simulink model "My_gfm_battery_sil_12_ConvIGBT_zDomain"  (R2025b)
settings: Solver=ode23t  StartTime=0.0  StopTime=10  MaxStep=1e-4  RelTol=1e-3
PreLoadFcn:
  | close all;
  | clear all;
  | clc;
  | 
  | 
  | modelDir = fileparts(get_param(bdroot,'FileName'));
  | 
  | load_system(fullfile(modelDir,'controls_element_lib.slx'));
  | load_system(fullfile(modelDir,'test_sequence_lib.slx'));
  | 
  | Simulink.importExternalCTypes('.\circuitControls\circuitControls_A_autogen.h')
InitFcn:
  | % frequency nominals
  | F_NOM = 60;
  | W_NOM = 2 * pi * F_NOM;
  | 
  | % base values relative to inverter
  | % --------------------------------
  | VLL_INV_NOM = 480;
  | P_INV_NOM = 1e6;
  | Q_INV_NOM = 0.5e6;
  | S_INV_NOM = sqrt(P_INV_NOM^2 + Q_INV_NOM^2);
  | 
  | I_INV_BASE = S_INV_NOM/(sqrt(3)*VLL_INV_NOM);
  | Z_INV_BASE = VLL_INV_NOM^2/S_INV_NOM;
  | L_INV_BASE = Z_INV_BASE / W_NOM;
  | C_INV_BASE = 1 / (Z_INV_BASE * W_NOM);
  | 
  | % nominal ratings for power system model
  | % --------------------------------------
  | INVERTER_COUNT = 100;
  | 
  | VLV_NOM = VLL_INV_NOM;
  | VMV_NOM = 35e3;
  | VHV_NOM = 230e3;
  | S_PLANT = INVERTER_COUNT * S_INV_NOM;
  | 
  | N_GSU = VHV_NOM/VMV_NOM;
  | N_MVT = VMV_NOM/VLV_NOM;
  | 
  | I_LV_BASE = S_PLANT/(sqrt(3)*VLV_NOM);
  | I_MV_BASE = S_PLANT/(sqrt(3)*VMV_NOM);
  | I_HV_BASE = S_PLANT/(sqrt(3)*VHV_NOM);
  | 
  | Z_LV_BASE = VLV_NOM^2/S_PLANT;
  | Z_MV_BASE = VMV_NOM^2/S_PLANT;
  | Z_HV_BASE = VHV_NOM^2/S_PLANT;
  | 
  | L_LV_BASE = Z_LV_BASE / W_NOM;
  | L_MV_BASE = Z_MV_BASE / W_NOM;
  | L_HV_BASE = Z_HV_BASE / W_NOM;
  | C_LV_BASE = 1 / (Z_LV_BASE * W_NOM);
  | C_MV_BASE = 1 / (Z_MV_BASE * W_NOM);
  | C_HV_BASE = 1 / (Z_HV_BASE * W_NOM);
undefined symbols (not defined in the file): D1, D11, Delta, gcbh, j, SampleTime, sps_rtmsupport, Ts
libraries: simulink x56, spsVoltageMeasurementLib x21, spsThreePhaseSeriesRLCBranchLib x20, spsControlledCurrentSourceLib x20, spsControlledVoltageSourceLib x15, spsThreePhaseVIMeasurementLib x12, spsSeriesRLCBranchLib x11, spsGroundLib x11, test_sequence_lib x10, controls_element_lib x8, spsCurrentMeasurementLib x8, spsThreePhaseTransformerTwoWindingsLib x6
(part 8 of 9)

== system My_gfm_battery_sil_12_ConvIGBT_zDomain/ac Network with MVT (native math)5/Network Interface1/CSI2 ==
  I : Inport
  Demux : Demux  Outputs=3
  Series RLC Branch : spsSeriesRLCBranchLib/Series RLC Branch  LConnTagsString=__new0  RConnTagsString=__new0  BranchType=R  Resistance=1e3  Inductance=1e-3  SetiL0=off  InitialCurrent=0  Capacitance=1e-6  Setx0=off  InitialVoltage=0  Measurements=None
  Series RLC Branch1 : spsSeriesRLCBranchLib/Series RLC Branch  LConnTagsString=__new0  RConnTagsString=__new0  BranchType=R  Resistance=1e3  Inductance=1e-3  SetiL0=off  InitialCurrent=0  Capacitance=1e-6  Setx0=off  InitialVoltage=0  Measurements=None
  Series RLC Branch2 : spsSeriesRLCBranchLib/Series RLC Branch  LConnTagsString=__new0  RConnTagsString=__new0  BranchType=R  Resistance=1e3  Inductance=1e-3  SetiL0=off  InitialCurrent=0  Capacitance=1e-6  Setx0=off  InitialVoltage=0  Measurements=None
  iA : spsControlledCurrentSourceLib/Controlled Current Source  Initialize=off  Source_Type=AC  Amplitude=0  Phase=0  Frequency=0  Measurements=None
  iB : spsControlledCurrentSourceLib/Controlled Current Source  Initialize=off  Source_Type=AC  Amplitude=0  Phase=0  Frequency=0  Measurements=None
  iB1 : spsControlledCurrentSourceLib/Controlled Current Source  Initialize=off  Source_Type=AC  Amplitude=0  Phase=0  Frequency=0  Measurements=None
  A : PMIOPort  Side=Right
  B : PMIOPort  Port=2  Side=Right
  C : PMIOPort  Port=3  Side=Right
  wires:
  Demux/1 -> iA/1
  Demux/2 -> iB/1
  I/1 -> Demux/1
  Demux/3 -> iB1/1
  connections:
  iA/RConn1 -- A/RConn1 -- Series RLC Branch/LConn1
  iB/RConn1 -- B/RConn1 -- Series RLC Branch1/LConn1
  Series RLC Branch1/RConn1 -- Series RLC Branch/RConn1 -- iA/LConn1 -- iB/LConn1 -- iB1/LConn1 -- Series RLC Branch2/RConn1
  C/RConn1 -- iB1/RConn1 -- Series RLC Branch2/LConn1

== system My_gfm_battery_sil_12_ConvIGBT_zDomain/ac Network with MVT (native math)5/Network Interface1/Cur Meas ==
  Current Measurement : spsCurrentMeasurementLib/Current Measurement  PhasorSimulation=off  OutputType=Complex  PSBequivalent=0
  Current Measurement1 : spsCurrentMeasurementLib/Current Measurement  PhasorSimulation=off  OutputType=Complex  PSBequivalent=0
  Current Measurement2 : spsCurrentMeasurementLib/Current Measurement  PhasorSimulation=off  OutputType=Complex  PSBequivalent=0
  Mux : Mux  Inputs=3
  A : PMIOPort  Side=Left
  B : PMIOPort  Port=2  Side=Left
  C : PMIOPort  Port=3  Side=Left
  a : PMIOPort  Port=4  Side=Right
  b : PMIOPort  Port=5  Side=Right
  c : PMIOPort  Port=6  Side=Right
  I : Outport  VectorParamsAs1DForOutWhenUnconnected=off
  wires:
  Current Measurement/1 -> Mux/1
  Current Measurement1/1 -> Mux/2
  Mux/1 -> I/1
  Current Measurement2/1 -> Mux/3
  connections:
  Current Measurement1/LConn1 -- B/RConn1
  Current Measurement/LConn1 -- A/RConn1
  Current Measurement2/LConn1 -- C/RConn1
  a/RConn1 -- Current Measurement/RConn1
  b/RConn1 -- Current Measurement1/RConn1
  c/RConn1 -- Current Measurement2/RConn1

== system My_gfm_battery_sil_12_ConvIGBT_zDomain/ac Network with MVT (native math)5/Network Interface1/Subsystem ==
  In1 : Inport
  Demux : Demux  Outputs=3
  Mux : Mux  Inputs=3
  Transfer Fcn : TransferFcn  Denominator=[1e-6 1]
  Transfer Fcn1 : TransferFcn  Denominator=[1e-6 1]
  Transfer Fcn2 : TransferFcn  Denominator=[1e-6 1]
  Out1 : Outport  VectorParamsAs1DForOutWhenUnconnected=off
  wires:
  Demux/2 -> Transfer Fcn2/1
  Demux/1 -> Transfer Fcn/1
  Transfer Fcn1/1 -> Mux/3
  Mux/1 -> Out1/1
  Transfer Fcn2/1 -> Mux/2
  Demux/3 -> Transfer Fcn1/1
  Transfer Fcn/1 -> Mux/1
  In1/1 -> Demux/1

== system My_gfm_battery_sil_12_ConvIGBT_zDomain/ac Network with MVT (native math)5/Network Interface1/Subsystem1 ==
  In1 : Inport
  Demux : Demux  Outputs=3
  Mux : Mux  Inputs=3
  Transfer Fcn : TransferFcn  Denominator=[1e-6 1]
  Transfer Fcn1 : TransferFcn  Denominator=[1e-6 1]
  Transfer Fcn2 : TransferFcn  Denominator=[1e-6 1]
  Out1 : Outport  VectorParamsAs1DForOutWhenUnconnected=off
  wires:
  Demux/2 -> Transfer Fcn2/1
  Demux/1 -> Transfer Fcn/1
  Transfer Fcn1/1 -> Mux/3
  Mux/1 -> Out1/1
  Transfer Fcn2/1 -> Mux/2
  Demux/3 -> Transfer Fcn1/1
  Transfer Fcn/1 -> Mux/1
  In1/1 -> Demux/1

== system My_gfm_battery_sil_12_ConvIGBT_zDomain/ac Network with MVT (native math)5/Network Interface1/VSI1 ==
  V : Inport
  Controlled Voltage Source : spsControlledVoltageSourceLib/Controlled Voltage Source  Initialize=off  Source_Type=AC  Amplitude=0  Phase=0  Frequency=0  Measurements=None
  Controlled Voltage Source1 : spsControlledVoltageSourceLib/Controlled Voltage Source  Initialize=off  Source_Type=AC  Amplitude=0  Phase=0  Frequency=0  Measurements=None
  Demux : Demux  Outputs=3
  Terminator : Terminator
  A : PMIOPort  Side=Right
  B : PMIOPort  Port=2  Side=Right
  C : PMIOPort  Port=3  Side=Right
  wires:
  Demux/1 -> Controlled Voltage Source/1
  Demux/2 -> Controlled Voltage Source1/1
  V/1 -> Demux/1
  Demux/3 -> Terminator/1
  connections:
  Controlled Voltage Source/RConn1 -- A/RConn1
  Controlled Voltage Source1/RConn1 -- B/RConn1
  Controlled Voltage Source1/LConn1 -- Controlled Voltage Source/LConn1 -- C/RConn1

== system My_gfm_battery_sil_12_ConvIGBT_zDomain/ac Network with MVT (native math)5/Network Interface1/Volt Meas1 ==
  Ground : Ground
  Mux : Mux  Inputs=3
  V_AB : spsVoltageMeasurementLib/Voltage Measurement  PhasorSimulation=off  OutputType=Complex  PSBequivalent=0
  V_BC : spsVoltageMeasurementLib/Voltage Measurement  PhasorSimulation=off  OutputType=Complex  PSBequivalent=0
  A : PMIOPort  Side=Left
  B : PMIOPort  Port=2  Side=Left
  C : PMIOPort  Port=3  Side=Left
  V : Outport  VectorParamsAs1DForOutWhenUnconnected=off
  wires:
  V_AB/1 -> Mux/1
  V_BC/1 -> Mux/2
  Mux/1 -> V/1  "[Vab,Vbc]"
  Ground/1 -> Mux/3
  connections:
  V_BC/LConn1 -- B/RConn1
  A/RConn1 -- V_AB/LConn1
  C/RConn1 -- V_AB/LConn2 -- V_BC/LConn2

== system My_gfm_battery_sil_12_ConvIGBT_zDomain/ac Network with MVT (native math)5/Two-Level Converter/Model1 ==
  note: (Uref)
  g : Inport  SampleTime=Ts
  Block : Inport  Port=2
  Add : Sum  Inputs=+-
  Constant : Constant
  Constant1 : Constant  Value=0
  Constant2 : Constant
  Current Measurement : spsCurrentMeasurementLib/Current Measurement  PhasorSimulation=off  OutputType=Complex  PSBequivalent=0
  Data Type Conversion2 : DataTypeConversion  OutDataTypeStr=double  SaturateOnIntegerOverflow=off  RndMeth=Floor
  Demux : Demux  Outputs=2
  Fcn2 : Fcn  Expr=(u(1)+1)*0.5
  MATLAB Function : MATLAB Function  TreatAsAtomicUnit=on
  Mux : Mux  Inputs=2
  Mux1 : Mux  Inputs=2
  Power : spsHalfBridgeModel/Power  SystemSampleTime=-1  VariantActivationTime=update diagram  EmptyChoice=off  PassThrough=off  PassThroughVariantControl=(default)  EmptyChoiceVariantControl=(default)  AllowFlexibleInterface=on  Latency=0  AutoFrameSizeCalculation=off
  Product2 : Product
  Product8 : Product
  Saturation : Saturate  UpperLimit=1.0  LowerLimit=-1.0
  Scope : Scope  NumInputPorts=2
      settings: ActiveDisplayYMinimum=-0.125  ActiveDisplayYMaximum=1.125
  Scope1 : Scope  NumInputPorts=2
      settings: ActiveDisplayYMinimum=0.0581  ActiveDisplayYMaximum=0.93277  DataLoggingVariableName=ScopeData2
  Scope2 : Scope  NumInputPorts=6
      settings: ActiveDisplayYMinimum=-1057.03298  ActiveDisplayYMaximum=1237.20421  DataLoggingVariableName=ScopeData3
  Switch : Switch  Criteria=u2 > Threshold  SaturateOnIntegerOverflow=off  InputSameDT=off
  Transfer Fcn : TransferFcn  Denominator=[1e-6 1]
  Transfer Fcn1 : TransferFcn  Denominator=[1e-6 1]
  Transfer Fcn2 : TransferFcn  Denominator=[1e-6 1]
  Voltage Measurement : spsVoltageMeasurementLib/Voltage Measurement  PhasorSimulation=off  OutputType=Complex  PSBequivalent=0
  + : PMIOPort  Tag=PMCPort  Side=Right
  - : PMIOPort  Tag=PMCPort  Port=2  Side=Right
  Out : PMIOPort  Tag=PMCPort  Port=3  Side=Left
  wires:
  Saturation/1 -> Fcn2/1
  g/1 -> Saturation/1
  Block/1 -> Switch/2, Scope/1
  Data Type Conversion2/1 -> Scope/2, Product2/1, Product8/1
  Product2/1 -> Mux1/1
  Product8/1 -> Mux1/2
  Add/1 -> Scope1/2, Product8/2
  Constant/1 -> Add/1
  Fcn2/1 -> Add/2, Scope1/1, Product2/2
  Switch/1 -> Data Type Conversion2/1
  Power/2 -> Scope2/4, Demux/1
  Demux/2 -> Transfer Fcn2/1
  Demux/1 -> Transfer Fcn/1
  Transfer Fcn/1 -> Mux/1
  Transfer Fcn2/1 -> Mux/2
  Mux/1 -> MATLAB Function/3(I)
  Transfer Fcn1/1 -> MATLAB Function/2(Vdc)
  Power/1 -> Scope2/2, Transfer Fcn1/1
  MATLAB Function/2(Idc) -> Power/2, Scope2/3
  MATLAB Function/1(V) -> Power/1, Scope2/1
  Mux1/1 -> MATLAB Function/1(g)
  Constant1/1 -> Switch/1
  Constant2/1 -> Switch/3
  Voltage Measurement/1 -> Scope2/5
  Current Measurement/1 -> Scope2/6
  connections:
  Power/LConn1 -- Current Measurement/LConn1 -- Voltage Measurement/LConn1
  Power/RConn2 -- Voltage Measurement/LConn2 -- -/RConn1
  Power/RConn1 -- +/RConn1
  Current Measurement/RConn1 -- Out/RConn1

== system My_gfm_battery_sil_12_ConvIGBT_zDomain/ac Network with MVT (native math)5/Two-Level Converter/Model2 ==
  note: (Uref)
  g : Inport  SampleTime=Ts
  Block : Inport  Port=2
  Add : Sum  Inputs=+-
  Constant : Constant
  Constant1 : Constant  Value=0
  Constant2 : Constant
  Data Type Conversion2 : DataTypeConversion  OutDataTypeStr=double  SaturateOnIntegerOverflow=off  RndMeth=Floor
  Demux : Demux  Outputs=2
  Fcn2 : Fcn  Expr=(u(1)+1)*0.5
  MATLAB Function : MATLAB Function  TreatAsAtomicUnit=on
  Mux : Mux  Inputs=2
  Mux1 : Mux  Inputs=2
  Power : spsHalfBridgeModel/Power  SystemSampleTime=-1  VariantActivationTime=update diagram  EmptyChoice=off  PassThrough=off  PassThroughVariantControl=(default)  EmptyChoiceVariantControl=(default)  AllowFlexibleInterface=on  Latency=0  AutoFrameSizeCalculation=off
  Product2 : Product
  Product8 : Product
  Saturation : Saturate  UpperLimit=1.0  LowerLimit=-1.0
  Scope : Scope  NumInputPorts=2
      settings: ActiveDisplayYMinimum=-0.125  ActiveDisplayYMaximum=1.125
  Scope1 : Scope  NumInputPorts=2
      settings: ActiveDisplayYMinimum=-0.0256  ActiveDisplayYMaximum=0.96024  DataLoggingVariableName=ScopeData2
  Scope2 : Scope  NumInputPorts=5
      settings: ActiveDisplayYMinimum=-1250  ActiveDisplayYMaximum=1079.00943  DataLoggingVariableName=ScopeData3
  Switch : Switch  Criteria=u2 > Threshold  SaturateOnIntegerOverflow=off  InputSameDT=off
  Transfer Fcn : TransferFcn  Denominator=[1e-6 1]
  Transfer Fcn1 : TransferFcn  Denominator=[1e-6 1]
  Transfer Fcn2 : TransferFcn  Denominator=[1e-6 1]
  Voltage Measurement : spsVoltageMeasurementLib/Voltage Measurement  PhasorSimulation=off  OutputType=Complex  PSBequivalent=0
  + : PMIOPort  Tag=PMCPort  Side=Right
  - : PMIOPort  Tag=PMCPort  Port=2  Side=Right
  Out : PMIOPort  Tag=PMCPort  Port=3  Side=Left
  wires:
  Saturation/1 -> Fcn2/1
  g/1 -> Saturation/1
  Block/1 -> Switch/2, Scope/1
  Data Type Conversion2/1 -> Scope/2, Product2/1, Product8/1
  Product2/1 -> Mux1/1
  Product8/1 -> Mux1/2
  Add/1 -> Scope1/2, Product8/2
  Constant/1 -> Add/1
  Fcn2/1 -> Add/2, Scope1/1, Product2/2
  Switch/1 -> Data Type Conversion2/1
  Power/2 -> Scope2/4, Demux/1
  Demux/2 -> Transfer Fcn2/1
  Demux/1 -> Transfer Fcn/1
  Transfer Fcn/1 -> Mux/1
  Transfer Fcn2/1 -> Mux/2
  Mux/1 -> MATLAB Function/3(I)
  Transfer Fcn1/1 -> MATLAB Function/2(Vdc)
  Power/1 -> Scope2/2, Transfer Fcn1/1
  MATLAB Function/2(Idc) -> Power/2, Scope2/3
  MATLAB Function/1(V) -> Power/1, Scope2/1
  Mux1/1 -> MATLAB Function/1(g)
  Constant1/1 -> Switch/1
  Constant2/1 -> Switch/3
  Voltage Measurement/1 -> Scope2/5
  connections:
  Out/RConn1 -- Power/LConn1 -- Voltage Measurement/LConn1
  -/RConn1 -- Power/RConn2 -- Voltage Measurement/LConn2
  Power/RConn1 -- +/RConn1

== system My_gfm_battery_sil_12_ConvIGBT_zDomain/ac Network with MVT (native math)5/Two-Level Converter/Model3 ==
  note: (Uref)
  g : Inport  SampleTime=Ts
  Block : Inport  Port=2
  Add : Sum  Inputs=+-
  Constant : Constant
  Constant1 : Constant  Value=0
  Constant2 : Constant
  Data Type Conversion2 : DataTypeConversion  OutDataTypeStr=double  SaturateOnIntegerOverflow=off  RndMeth=Floor
  Demux : Demux  Outputs=2
  Fcn2 : Fcn  Expr=(u(1)+1)*0.5
  MATLAB Function : MATLAB Function  TreatAsAtomicUnit=on
  Mux : Mux  Inputs=2
  Mux1 : Mux  Inputs=2
  Power : spsHalfBridgeModel/Power  SystemSampleTime=-1  VariantActivationTime=update diagram  EmptyChoice=off  PassThrough=off  PassThroughVariantControl=(default)  EmptyChoiceVariantControl=(default)  AllowFlexibleInterface=on  Latency=0  AutoFrameSizeCalculation=off
  Product2 : Product
  Product8 : Product
  Saturation : Saturate  UpperLimit=1.0  LowerLimit=-1.0
  Scope : Scope  NumInputPorts=2
      settings: ActiveDisplayYMinimum=-0.125  ActiveDisplayYMaximum=1.125
  Scope1 : Scope  NumInputPorts=2
      settings: ActiveDisplayYMinimum=-0.0256  ActiveDisplayYMaximum=0.96024  DataLoggingVariableName=ScopeData2
  Scope2 : Scope  NumInputPorts=5
      settings: ActiveDisplayYMinimum=-1250  ActiveDisplayYMaximum=1079.00943  DataLoggingVariableName=ScopeData3
  Switch : Switch  Criteria=u2 > Threshold  SaturateOnIntegerOverflow=off  InputSameDT=off
  Transfer Fcn : TransferFcn  Denominator=[1e-6 1]
  Transfer Fcn1 : TransferFcn  Denominator=[1e-6 1]
  Transfer Fcn2 : TransferFcn  Denominator=[1e-6 1]
  Voltage Measurement : spsVoltageMeasurementLib/Voltage Measurement  PhasorSimulation=off  OutputType=Complex  PSBequivalent=0
  + : PMIOPort  Tag=PMCPort  Side=Right
  - : PMIOPort  Tag=PMCPort  Port=2  Side=Right
  Out : PMIOPort  Tag=PMCPort  Port=3  Side=Left
  wires:
  Saturation/1 -> Fcn2/1
  g/1 -> Saturation/1
  Block/1 -> Switch/2, Scope/1
  Data Type Conversion2/1 -> Scope/2, Product2/1, Product8/1
  Product2/1 -> Mux1/1
  Product8/1 -> Mux1/2
  Add/1 -> Scope1/2, Product8/2
  Constant/1 -> Add/1
  Fcn2/1 -> Add/2, Scope1/1, Product2/2
  Switch/1 -> Data Type Conversion2/1
  Power/2 -> Scope2/4, Demux/1
  Demux/2 -> Transfer Fcn2/1
  Demux/1 -> Transfer Fcn/1
  Transfer Fcn/1 -> Mux/1
  Transfer Fcn2/1 -> Mux/2
  Mux/1 -> MATLAB Function/3(I)
  Transfer Fcn1/1 -> MATLAB Function/2(Vdc)
  Power/1 -> Scope2/2, Transfer Fcn1/1
  MATLAB Function/2(Idc) -> Power/2, Scope2/3
  MATLAB Function/1(V) -> Power/1, Scope2/1
  Mux1/1 -> MATLAB Function/1(g)
  Constant1/1 -> Switch/1
  Constant2/1 -> Switch/3
  Voltage Measurement/1 -> Scope2/5
  connections:
  Out/RConn1 -- Power/LConn1 -- Voltage Measurement/LConn1
  -/RConn1 -- Power/RConn2 -- Voltage Measurement/LConn2
  Power/RConn1 -- +/RConn1

== system My_gfm_battery_sil_12_ConvIGBT_zDomain/My Inverter Controller /My_acMonitor_A/Analyzer_V/complex_LPF ==
  note: This was needed because Simulink complains when using transfer functions directly on arrays or complex numbers.
  In1 : Inport
  Complex to Real-Imag : ComplexToRealImag
  LPF1 : Subsystem  SystemSampleTime=1/20000  mask(Low Pass Filter){Ts=Ts, OmegaUp=1/tau, OmegaDn=1/tau}
      mask prompts: Ts "Tsample"; OmegaUp "Up Path Bandwidth"; OmegaDn "Down Path Bandwidth"
  LPF4 : Subsystem  SystemSampleTime=1/20000  mask(Low Pass Filter){Ts=Ts, OmegaUp=1/tau, OmegaDn=1/tau}
      mask prompts: Ts "Tsample"; OmegaUp "Up Path Bandwidth"; OmegaDn "Down Path Bandwidth"
  Real-Imag to Complex : RealImagToComplex
  Out1 : Outport
  wires:
  Real-Imag to Complex/1 -> Out1/1
  In1/1 -> Complex to Real-Imag/1
  Complex to Real-Imag/1 -> LPF4/1(in)
  LPF4/1(out) -> Real-Imag to Complex/1
  Complex to Real-Imag/2 -> LPF1/1(in)
  LPF1/1(out) -> Real-Imag to Complex/2

== system My_gfm_battery_sil_12_ConvIGBT_zDomain/My Inverter Controller /My_acMonitor_A/Analyzer_V1/complex_LPF ==
  note: This was needed because Simulink complains when using transfer functions directly on arrays or complex numbers.
  In1 : Inport
  Complex to Real-Imag : ComplexToRealImag
  Gain2 : Gain  Gain=1/tau
  Gain3 : Gain  Gain=1/tau
  Integrator : Integrator
  Integrator1 : Integrator
  Real-Imag to Complex : RealImagToComplex
  Sum : Sum  Inputs=|+-
  Sum1 : Sum  Inputs=|+-
  Out1 : Outport
  wires:
  Real-Imag to Complex/1 -> Out1/1
  In1/1 -> Complex to Real-Imag/1
  Complex to Real-Imag/1 -> Sum/1
  Integrator/1 -> Real-Imag to Complex/1, Sum/2
  Sum1/1 -> Gain3/1
  Complex to Real-Imag/2 -> Sum1/1
  Gain2/1 -> Integrator/1
  Sum/1 -> Gain2/1
  Integrator1/1 -> Sum1/2, Real-Imag to Complex/2
  Gain3/1 -> Integrator1/1

== system My_gfm_battery_sil_12_ConvIGBT_zDomain/My Inverter Controller /My_acMonitor_A/PLL_3ph1/Integrator ==
  in : Inport
  rst : Inport  Port=2
  Constant : Constant  Value=0
  Constant1 : Constant  Value=HiLim
  Constant2 : Constant  Value=LoLim
  Constant3 : Constant  Value=Ts
  Delay : Delay  DelayLength=1  InitialCondition=0
  Logical Operator : Logic  Operator=NOT  AllPortsSameDT=off  OutDataTypeStr=boolean
  Product : Product
  Saturation Dynamic : simulink/Discontinuities/Saturation Dynamic  OutMin=[]  OutMax=[]  OutDataTypeStr=Inherit: Same as second input  OutDataType=fixdt(1, 16)  OutScaling=2^-10  DoSatur=off
  Sum : Sum  Inputs=|++
  Switch : Switch  Criteria=u2 ~= 0  SaturateOnIntegerOverflow=off  InputSameDT=off
  out : Outport
  FB : Outport  Port=2
  wires:
  Delay/1 -> Sum/2, FB/1
  Switch/1 -> Saturation Dynamic/2
  in/1 -> Product/2
  Product/1 -> Sum/1
  Constant3/1 -> Product/1
  Sum/1 -> Switch/1
  Constant/1 -> Switch/3
  rst/1 -> Logical Operator/1
  Logical Operator/1 -> Switch/2
  Saturation Dynamic/1 -> out/1, Delay/1
  Constant1/1 -> Saturation Dynamic/1
  Constant2/1 -> Saturation Dynamic/3

== system My_gfm_battery_sil_12_ConvIGBT_zDomain/My Inverter Controller /My_acMonitor_A/PLL_3ph1/LPF4 ==
  note: Forward integrator
  in : Inport
  Constant : Constant  Value=Ts
  Constant1 : Constant  Value=Ts
  Constant2 : Constant  Value=OmegaUp
  Constant3 : Constant  Value=OmegaUp
  Constant4 : Constant  Value=OmegaDn
  Delay : Delay  DelayLength=1  InitialCondition=0
  Product{,1..4} (5 alike) : Product
  Saturation : Saturate  UpperLimit=inf  LowerLimit=0
  Saturation1 : Saturate  UpperLimit=0  LowerLimit=-inf
  Sum : Sum  Inputs=|++
  Sum1 : Sum  Inputs=|++
  Sum4 : Sum  Inputs=|+-
  out : Outport
  wires:
  Delay/1 -> Sum4/2, Sum/2
  in/1 -> Sum4/1, Product4/2
  Sum4/1 -> Product2/1, Product1/2
  Sum/1 -> out/1, Delay/1
  Saturation/1 -> Sum1/1
  Saturation1/1 -> Sum1/2
  Sum1/1 -> Product/2
  Product/1 -> Sum/1
  Constant/1 -> Product/1
  Constant3/1 -> Product1/1
  Constant4/1 -> Product2/2
  Product1/1 -> Saturation/1
  Product2/1 -> Saturation1/1
  Product4/1 -> Product3/2
  Constant1/1 -> Product3/1
  Constant2/1 -> Product4/1

== system My_gfm_battery_sil_12_ConvIGBT_zDomain/My Inverter Controller /My_acMonitor_A/PLL_3ph1/SOGI1 ==
  in : Inport
  f : Inport  Port=2
  Gain : Gain
  Gain1 : Gain  Gain=alpha
  Gain2 : Gain  Gain=2*pi
  Ground : Ground
  Ground1 : Ground
  Integrator : Subsystem  SystemSampleTime=1/20000  mask(Limited Integrator){Ts=Ts, HiLim=inf, LoLim=-inf}
      mask prompts: Ts "Tsample"; HiLim "Integrator Upper Limiter"; LoLim "Integrator Lower Limiter"
  Integrator1 : Subsystem  SystemSampleTime=1/20000  mask(Limited Integrator){Ts=Ts, HiLim=inf, LoLim=-inf}
      mask prompts: Ts "Tsample"; HiLim "Integrator Upper Limiter"; LoLim "Integrator Lower Limiter"
  Product : Product
  Product2 : Product
  Sum : Sum  Inputs=|+-
  Sum1 : Sum  Inputs=|+-
  Sum2 : Sum  Inputs=|+-
  Terminator : Terminator
  Notched : Outport
  BandPassed : Outport  Port=2
  wires:
  f/1 -> Gain2/1
  in/1 -> Sum2/1, Sum1/1
  Integrator1/2(FB) -> Product2/1
  Gain/1 -> Sum1/2
  Sum1/1 -> Gain1/1
  Integrator/1(out) -> Integrator1/1(in), BandPassed/1
  Gain2/1 -> Product/2, Product2/2
  Sum/1 -> Product/1
  Product2/1 -> Sum/2
  Product/1 -> Integrator/1(in)
  Integrator/2(FB) -> Sum2/2, Gain/1
  Sum2/1 -> Notched/1
  Ground/1 -> Integrator/2(rst)
  Ground1/1 -> Integrator1/2(rst)
  Integrator1/1(out) -> Terminator/1
  Gain1/1 -> Sum/1

== system My_gfm_battery_sil_12_ConvIGBT_zDomain/My Inverter Controller /My_acMonitor_A/PLL_3ph1/oscillator_3ph ==
  f : Inport
  Cos : Trigonometry  Operator=cos
  Delay : Delay  DelayLength=1  InitialCondition=0
  Gain : Gain  Gain=2*pi
  Ground1 : Ground
  Integrator : Subsystem  SystemSampleTime=1/20000  mask(Wrapped Integrator){Ts=Ts}
      mask prompts: Ts "Tsample"
      mask help: output range : [0 to 1]
  Real-Imag to Complex : RealImagToComplex
  Scope : Scope
      settings: ActiveDisplayYMinimum=-0.026446027315415011  ActiveDisplayYMaximum=1.0606778639513765  DataLoggingVariableName=ScopeData13
  Sin : Trigonometry
  Sum1 : Sum  Inputs=|++
  Terminator : Terminator
  phase_shift : Constant  Value=[0 -1/3 -2/3]
  osc[3] : Outport
  osc[3]_FB : Outport  Port=2
  wires:
  Sum1/1 -> Gain/1
  phase_shift/1 -> Sum1/2
  Sin/1 -> Real-Imag to Complex/2
  Gain/1 -> Sin/1, Cos/1
  Cos/1 -> Real-Imag to Complex/1
  Real-Imag to Complex/1 -> Delay/1, osc[3]/1
  f/1 -> Integrator/1(in)
  Delay/1 -> osc[3]_FB/1
  Integrator/2(FB) -> Terminator/1
  Ground1/1 -> Integrator/2(rst)
  Integrator/1(out) -> Scope/1, Sum1/1

== system My_gfm_battery_sil_12_ConvIGBT_zDomain/My Inverter Controller /My_acMonitor_A/PLL_3ph2/oscillator_3ph ==
  f : Inport
  Cos : Trigonometry  Operator=cos
  Gain : Gain  Gain=2*pi
  Integrator : Integrator
  Real-Imag to Complex : RealImagToComplex
  Sin : Trigonometry
  Sum1 : Sum  Inputs=|++
  phase_shift : Constant  Value=[0 -1/3 -2/3]
  osc[3] : Outport
  wires:
  Sum1/1 -> Gain/1
  phase_shift/1 -> Sum1/2
  Sin/1 -> Real-Imag to Complex/2
  Integrator/1 -> Sum1/1
  Gain/1 -> Sin/1, Cos/1
  Cos/1 -> Real-Imag to Complex/1
  Real-Imag to Complex/1 -> osc[3]/1
  f/1 -> Integrator/1

== system My_gfm_battery_sil_12_ConvIGBT_zDomain/My Inverter Controller /My_acMonitor_A/RMS_Analyzer/LPF4 ==
  note: Forward integrator
  in : Inport
  Constant : Constant  Value=Ts
  Constant1 : Constant  Value=Ts
  Constant2 : Constant  Value=OmegaUp
  Constant3 : Constant  Value=OmegaUp
  Constant4 : Constant  Value=OmegaDn
  Delay : Delay  DelayLength=1  InitialCondition=0
  Product{,1..4} (5 alike) : Product
  Saturation : Saturate  UpperLimit=inf  LowerLimit=0
  Saturation1 : Saturate  UpperLimit=0  LowerLimit=-inf
  Sum : Sum  Inputs=|++
  Sum1 : Sum  Inputs=|++
  Sum4 : Sum  Inputs=|+-
  out : Outport
  wires:
  Delay/1 -> Sum4/2, Sum/2
  in/1 -> Sum4/1, Product4/2
  Sum4/1 -> Product2/1, Product1/2
  Sum/1 -> out/1, Delay/1
  Saturation/1 -> Sum1/1
  Saturation1/1 -> Sum1/2
  Sum1/1 -> Product/2
  Product/1 -> Sum/1
  Constant/1 -> Product/1
  Constant3/1 -> Product1/1
  Constant4/1 -> Product2/2
  Product1/1 -> Saturation/1
  Product2/1 -> Saturation1/1
  Product4/1 -> Product3/2
  Constant1/1 -> Product3/1
  Constant2/1 -> Product4/1

== system My_gfm_battery_sil_12_ConvIGBT_zDomain/My Inverter Controller /My_acMonitor_A/SOGI1/Integrator ==
  in : Inport
  rst : Inport  Port=2
  Constant : Constant  Value=0
  Constant1 : Constant  Value=HiLim
  Constant2 : Constant  Value=LoLim
  Constant3 : Constant  Value=Ts
  Delay : Delay  DelayLength=1  InitialCondition=0
  Logical Operator : Logic  Operator=NOT  AllPortsSameDT=off  OutDataTypeStr=boolean
  Product : Product
  Saturation Dynamic : simulink/Discontinuities/Saturation Dynamic  OutMin=[]  OutMax=[]  OutDataTypeStr=Inherit: Same as second input  OutDataType=fixdt(1, 16)  OutScaling=2^-10  DoSatur=off
  Sum : Sum  Inputs=|++
  Switch : Switch  Criteria=u2 ~= 0  SaturateOnIntegerOverflow=off  InputSameDT=off
  out : Outport
  FB : Outport  Port=2
  wires:
  Delay/1 -> Sum/2, FB/1
  Switch/1 -> Saturation Dynamic/2
  in/1 -> Product/2
  Product/1 -> Sum/1
  Constant3/1 -> Product/1
  Sum/1 -> Switch/1
  Constant/1 -> Switch/3
  rst/1 -> Logical Operator/1
  Logical Operator/1 -> Switch/2
  Saturation Dynamic/1 -> out/1, Delay/1
  Constant1/1 -> Saturation Dynamic/1
  Constant2/1 -> Saturation Dynamic/3

== system My_gfm_battery_sil_12_ConvIGBT_zDomain/My Inverter Controller /My_acMonitor_A/SOGI1/Integrator1 ==
  in : Inport
  rst : Inport  Port=2
  Constant : Constant  Value=0
  Constant1 : Constant  Value=HiLim
  Constant2 : Constant  Value=LoLim
  Constant3 : Constant  Value=Ts
  Delay : Delay  DelayLength=1  InitialCondition=0
  Logical Operator : Logic  Operator=NOT  AllPortsSameDT=off  OutDataTypeStr=boolean
  Product : Product
  Saturation Dynamic : simulink/Discontinuities/Saturation Dynamic  OutMin=[]  OutMax=[]  OutDataTypeStr=Inherit: Same as second input  OutDataType=fixdt(1, 16)  OutScaling=2^-10  DoSatur=off
  Sum : Sum  Inputs=|++
  Switch : Switch  Criteria=u2 ~= 0  SaturateOnIntegerOverflow=off  InputSameDT=off
  out : Outport
  FB : Outport  Port=2
  wires:
  Delay/1 -> Sum/2, FB/1
  Switch/1 -> Saturation Dynamic/2
  in/1 -> Product/2
  Product/1 -> Sum/1
  Constant3/1 -> Product/1
  Sum/1 -> Switch/1
  Constant/1 -> Switch/3
  rst/1 -> Logical Operator/1
  Logical Operator/1 -> Switch/2
  Saturation Dynamic/1 -> out/1, Delay/1
  Constant1/1 -> Saturation Dynamic/1
  Constant2/1 -> Saturation Dynamic/3

== system My_gfm_battery_sil_12_ConvIGBT_zDomain/My Inverter Controller /My_acMonitor_A1/Analyzer_V/complex_LPF ==
  note: This was needed because Simulink complains when using transfer functions directly on arrays or complex numbers.
  In1 : Inport
  Complex to Real-Imag : ComplexToRealImag
  Gain2 : Gain  Gain=1/tau
  Gain3 : Gain  Gain=1/tau
  Integrator : Integrator
  Integrator1 : Integrator
  Real-Imag to Complex : RealImagToComplex
  Sum : Sum  Inputs=|+-
  Sum1 : Sum  Inputs=|+-
  Out1 : Outport
  wires:
  Real-Imag to Complex/1 -> Out1/1
  In1/1 -> Complex to Real-Imag/1
  Complex to Real-Imag/1 -> Sum/1
  Integrator/1 -> Real-Imag to Complex/1, Sum/2
  Sum1/1 -> Gain3/1
  Complex to Real-Imag/2 -> Sum1/1
  Gain2/1 -> Integrator/1
  Sum/1 -> Gain2/1
  Integrator1/1 -> Sum1/2, Real-Imag to Complex/2
  Gain3/1 -> Integrator1/1

== system My_gfm_battery_sil_12_ConvIGBT_zDomain/My Inverter Controller /My_acMonitor_A1/Analyzer_V1/complex_LPF ==
  note: This was needed because Simulink complains when using transfer functions directly on arrays or complex numbers.
  In1 : Inport
  Complex to Real-Imag : ComplexToRealImag
  Gain2 : Gain  Gain=1/tau
  Gain3 : Gain  Gain=1/tau
  Integrator : Integrator
  Integrator1 : Integrator
  Real-Imag to Complex : RealImagToComplex
  Sum : Sum  Inputs=|+-
  Sum1 : Sum  Inputs=|+-
  Out1 : Outport
  wires:
  Real-Imag to Complex/1 -> Out1/1
  In1/1 -> Complex to Real-Imag/1
  Complex to Real-Imag/1 -> Sum/1
  Integrator/1 -> Real-Imag to Complex/1, Sum/2
  Sum1/1 -> Gain3/1
  Complex to Real-Imag/2 -> Sum1/1
  Gain2/1 -> Integrator/1
  Sum/1 -> Gain2/1
  Integrator1/1 -> Sum1/2, Real-Imag to Complex/2
  Gain3/1 -> Integrator1/1

== system My_gfm_battery_sil_12_ConvIGBT_zDomain/My Inverter Controller /My_acMonitor_A1/PLL_3ph/oscillator_3ph ==
  f : Inport
  Cos : Trigonometry  Operator=cos
  Gain : Gain  Gain=2*pi
  Integrator : Integrator
  Real-Imag to Complex : RealImagToComplex
  Sin : Trigonometry
  Sum1 : Sum  Inputs=|++
  phase_shift : Constant  Value=[0 -1/3 -2/3]
  osc[3] : Outport
  wires:
  Sum1/1 -> Gain/1
  phase_shift/1 -> Sum1/2
  Sin/1 -> Real-Imag to Complex/2
  Integrator/1 -> Sum1/1
  Gain/1 -> Sin/1, Cos/1
  Cos/1 -> Real-Imag to Complex/1
  Real-Imag to Complex/1 -> osc[3]/1
  f/1 -> Integrator/1

== system My_gfm_battery_sil_12_ConvIGBT_zDomain/My Inverter Controller /My_circuit_controls_A2/SOGI/Integrator1 ==
  In : Inport
  Ts : Inport  Port=2
  Delay1 : Delay  DelayLength=1
  Delay2 : Delay  DelayLength=1
  Delay3 : Delay  DelayLength=1
  Gain : Gain  Gain=1/12
  Gain1 : Gain  Gain=23
  Gain2 : Gain  Gain=16
  Gain3 : Gain  Gain=5
  Product : Product
  Sum : Sum  Inputs=|+-
  Sum1 : Sum  Inputs=|++
  Sum2 : Sum  Inputs=|++
  Out : Outport  VectorParamsAs1DForOutWhenUnconnected=off
  wires:
  Delay2/1 -> Gain2/1, Delay3/1
  Delay1/1 -> Sum2/2, Gain1/1, Delay2/1
  Delay3/1 -> Gain3/1
  Gain2/1 -> Sum/2
  Gain1/1 -> Sum/1
  Gain3/1 -> Sum1/2
  Sum/1 -> Sum1/1
  Gain/1 -> Sum2/1
  Sum2/1 -> Delay1/1
  Product/1 -> Gain/1
  Sum1/1 -> Out/1
  Ts/1 -> Product/2
  In/1 -> Product/1

== system My_gfm_battery_sil_12_ConvIGBT_zDomain/My Inverter Controller /My_circuit_controls_A2/SOGI/Integrator3 ==
  In : Inport
  Ts : Inport  Port=2
  Delay1 : Delay  DelayLength=1
  Delay2 : Delay  DelayLength=1
  Delay3 : Delay  DelayLength=1
  Gain : Gain  Gain=1/12
  Gain1 : Gain  Gain=23
  Gain2 : Gain  Gain=16
  Gain3 : Gain  Gain=5
  Product : Product
  Sum : Sum  Inputs=|+-
  Sum1 : Sum  Inputs=|++
  Sum2 : Sum  Inputs=|++
  Out : Outport  VectorParamsAs1DForOutWhenUnconnected=off
  wires:
  Delay2/1 -> Gain2/1, Delay3/1
  Delay1/1 -> Sum2/2, Gain1/1, Delay2/1
  Delay3/1 -> Gain3/1
  Gain2/1 -> Sum/2
  Gain1/1 -> Sum/1
  Gain3/1 -> Sum1/2
  Sum/1 -> Sum1/1
  Gain/1 -> Sum2/1
  Sum2/1 -> Delay1/1
  Product/1 -> Gain/1
  Sum1/1 -> Out/1
  Ts/1 -> Product/2
  In/1 -> Product/1

== system My_gfm_battery_sil_12_ConvIGBT_zDomain/My Inverter Controller /My_circuit_controls_A2/SOGI1/Integrator ==
  in : Inport
  rst : Inport  Port=2
  Constant : Constant  Value=0
  Constant1 : Constant  Value=Ts
  Delay : Delay  DelayLength=1  InitialCondition=0
  Logical Operator : Logic  Operator=NOT  AllPortsSameDT=off  OutDataTypeStr=boolean
  Product : Product
  Sum : Sum  Inputs=|++
  Switch : Switch  Criteria=u2 ~= 0  SaturateOnIntegerOverflow=off  InputSameDT=off
  out : Outport
  FB : Outport  Port=2
  wires:
  Delay/1 -> Sum/2, FB/1
  Switch/1 -> out/1, Delay/1
  in/1 -> Product/2
  Product/1 -> Sum/1
  Constant1/1 -> Product/1
  Sum/1 -> Switch/1
  Constant/1 -> Switch/3
  rst/1 -> Logical Operator/1
  Logical Operator/1 -> Switch/2

== system My_gfm_battery_sil_12_ConvIGBT_zDomain/My Inverter Controller /My_circuit_controls_A2/SOGI1/Integrator1 ==
  in : Inport
  rst : Inport  Port=2
  Constant : Constant  Value=0
  Constant1 : Constant  Value=Ts
  Delay : Delay  DelayLength=1  InitialCondition=0
  Logical Operator : Logic  Operator=NOT  AllPortsSameDT=off  OutDataTypeStr=boolean
  Product : Product
  Sum : Sum  Inputs=|++
  Switch : Switch  Criteria=u2 ~= 0  SaturateOnIntegerOverflow=off  InputSameDT=off
  out : Outport
  FB : Outport  Port=2
  wires:
  Delay/1 -> Sum/2, FB/1
  Switch/1 -> out/1, Delay/1
  in/1 -> Product/2
  Product/1 -> Sum/1
  Constant1/1 -> Product/1
  Sum/1 -> Switch/1
  Constant/1 -> Switch/3
  rst/1 -> Logical Operator/1
  Logical Operator/1 -> Switch/2

== system My_gfm_battery_sil_12_ConvIGBT_zDomain/My Inverter Controller /My_circuit_controls_A2/Subsystem/LPF4 ==
  note: Forward integrator
  in : Inport
  Constant2 : Constant  Value=Ts
  Constant3 : Constant  Value=OmegaUp
  Constant4 : Constant  Value=OmegaDn
  Constant9 : Constant  Value=1/20000
  Delay : Delay  DelayLength=1  InitialCondition=0
  Gain : Gain  Gain=1/5
  Math Function : Math  Operator=reciprocal  SignedPower=on
  MinMax : MinMax  Function=max  Inputs=2
  MinMax1 : MinMax  Inputs=2
  MinMax2 : MinMax  Inputs=2
  Product : Product
  Product1 : Product
  Product2 : Product
  Saturation : Saturate  UpperLimit=inf  LowerLimit=0
  Saturation1 : Saturate  UpperLimit=0  LowerLimit=-inf
  Sum : Sum  Inputs=|++
  Sum1 : Sum  Inputs=|++
  Sum4 : Sum  Inputs=|+-
  out : Outport
  wires:
  Delay/1 -> Sum4/2, Sum/2
  in/1 -> Sum4/1
  Sum4/1 -> Product2/1, Product1/2
  Sum/1 -> out/1, Delay/1
  Saturation/1 -> Sum1/1
  Saturation1/1 -> Sum1/2
  Sum1/1 -> Product/2
  Product/1 -> Sum/1
  [Ts] -> Product/1
  [OmegaUp] -> Product1/1
  [OmegaDn] -> Product2/2
  Constant2/1 -> MinMax/1
  MinMax/1 -> [Ts]
  Constant9/1 -> MinMax/2
  MinMax1/1 -> [OmegaUp]
  MinMax2/1 -> [OmegaDn]
  [Ts] -> Math Function/1
  Math Function/1 -> Gain/1
  Gain/1 -> MinMax1/2, MinMax2/1
  Constant3/1 -> MinMax1/1
  Constant4/1 -> MinMax2/2
  Product1/1 -> Saturation/1
  Product2/1 -> Saturation1/1

== system My_gfm_battery_sil_12_ConvIGBT_zDomain/My Inverter Controller /My_circuit_controls_A2/virtual damper/Damping HPF ==
  note: Forward integrator
  in : Inport
  Constant2 : Constant  Value=Ts
  Constant3 : Constant  Value=OmegaUp
  Constant4 : Constant  Value=OmegaDn
  Constant9 : Constant  Value=1/20000
  Delay : Delay  DelayLength=1  InitialCondition=0
  Gain : Gain  Gain=1/5
  Math Function : Math  Operator=reciprocal  SignedPower=on
  MinMax : MinMax  Function=max  Inputs=2
  MinMax1 : MinMax  Inputs=2
  MinMax2 : MinMax  Inputs=2
  Product : Product
  Product1 : Product
  Product2 : Product
  Saturation : Saturate  UpperLimit=inf  LowerLimit=0
  Saturation1 : Saturate  UpperLimit=0  LowerLimit=-inf
  Sum : Sum  Inputs=|+-
  Sum1 : Sum  Inputs=|++
  Sum2 : Sum  Inputs=|++
  Sum3 : Sum  Inputs=|+-
  out : Outport  VectorParamsAs1DForOutWhenUnconnected=off
  wires:
  Gain/1 -> MinMax1/2, MinMax2/1
  [Ts] -> Product/1
  [Ts] -> Math Function/1
  Delay/1 -> Sum1/2, Sum/2
  MinMax1/1 -> [OmegaUp]
  Constant9/1 -> MinMax/2
  Sum/1 -> Product2/1, Product1/2
  Math Function/1 -> Gain/1
  Constant4/1 -> MinMax2/2
  Constant2/1 -> MinMax/1
  Saturation/1 -> Sum2/1
  Sum1/1 -> Sum3/2, Delay/1
  Sum2/1 -> Product/2
  MinMax2/1 -> [OmegaDn]
  Product/1 -> Sum1/1
  [OmegaUp] -> Product1/1
  Constant3/1 -> MinMax1/1
  MinMax/1 -> [Ts]
  Product2/1 -> Saturation1/1
  in/1 -> Sum3/1, Sum/1
  Product1/1 -> Saturation/1
  [OmegaDn] -> Product2/2
  Saturation1/1 -> Sum2/2
  Sum3/1 -> out/1

== system My_gfm_battery_sil_12_ConvIGBT_zDomain/My Inverter Controller /My_circuit_controls_A4/SOGI/Integrator1 ==
  In : Inport
  Ts : Inport  Port=2
  Delay1 : Delay  DelayLength=1
  Delay2 : Delay  DelayLength=1
  Delay3 : Delay  DelayLength=1
  Gain : Gain  Gain=1/12
  Gain1 : Gain  Gain=23
  Gain2 : Gain  Gain=16
  Gain3 : Gain  Gain=5
  Product : Product
  Sum : Sum  Inputs=|+-
  Sum1 : Sum  Inputs=|++
  Sum2 : Sum  Inputs=|++
  Out : Outport  VectorParamsAs1DForOutWhenUnconnected=off
  wires:
  Delay2/1 -> Gain2/1, Delay3/1
  Delay1/1 -> Sum2/2, Gain1/1, Delay2/1
  Delay3/1 -> Gain3/1
  Gain2/1 -> Sum/2
  Gain1/1 -> Sum/1
  Gain3/1 -> Sum1/2
  Sum/1 -> Sum1/1
  Gain/1 -> Sum2/1
  Sum2/1 -> Delay1/1
  Product/1 -> Gain/1
  Sum1/1 -> Out/1
  Ts/1 -> Product/2
  In/1 -> Product/1

== system My_gfm_battery_sil_12_ConvIGBT_zDomain/My Inverter Controller /My_circuit_controls_A4/SOGI/Integrator3 ==
  In : Inport
  Ts : Inport  Port=2
  Delay1 : Delay  DelayLength=1
  Delay2 : Delay  DelayLength=1
  Delay3 : Delay  DelayLength=1
  Gain : Gain  Gain=1/12
  Gain1 : Gain  Gain=23
  Gain2 : Gain  Gain=16
  Gain3 : Gain  Gain=5
  Product : Product
  Sum : Sum  Inputs=|+-
  Sum1 : Sum  Inputs=|++
  Sum2 : Sum  Inputs=|++
  Out : Outport  VectorParamsAs1DForOutWhenUnconnected=off
  wires:
  Delay2/1 -> Gain2/1, Delay3/1
  Delay1/1 -> Sum2/2, Gain1/1, Delay2/1
  Delay3/1 -> Gain3/1
  Gain2/1 -> Sum/2
  Gain1/1 -> Sum/1
  Gain3/1 -> Sum1/2
  Sum/1 -> Sum1/1
  Gain/1 -> Sum2/1
  Sum2/1 -> Delay1/1
  Product/1 -> Gain/1
  Sum1/1 -> Out/1
  Ts/1 -> Product/2
  In/1 -> Product/1

== system My_gfm_battery_sil_12_ConvIGBT_zDomain/My Inverter Controller /My_circuit_controls_A4/Subsystem/LPF4 ==
  note: Forward integrator
  in : Inport
  Constant2 : Constant  Value=Ts
  Constant3 : Constant  Value=OmegaUp
  Constant4 : Constant  Value=OmegaDn
  Constant9 : Constant  Value=1/20000
  Delay : Delay  DelayLength=1  InitialCondition=0
  Gain : Gain  Gain=1/5
  Math Function : Math  Operator=reciprocal  SignedPower=on
  MinMax : MinMax  Function=max  Inputs=2
  MinMax1 : MinMax  Inputs=2
  MinMax2 : MinMax  Inputs=2
  Product : Product
  Product1 : Product
  Product2 : Product
  Saturation : Saturate  UpperLimit=inf  LowerLimit=0
  Saturation1 : Saturate  UpperLimit=0  LowerLimit=-inf
  Sum : Sum  Inputs=|++
  Sum1 : Sum  Inputs=|++
  Sum4 : Sum  Inputs=|+-
  out : Outport
  wires:
  Delay/1 -> Sum4/2, Sum/2
  in/1 -> Sum4/1
  Sum4/1 -> Product2/1, Product1/2
  Sum/1 -> out/1, Delay/1
  Saturation/1 -> Sum1/1
  Saturation1/1 -> Sum1/2
  Sum1/1 -> Product/2
  Product/1 -> Sum/1
  [Ts] -> Product/1
  [OmegaUp] -> Product1/1
  [OmegaDn] -> Product2/2
  Constant2/1 -> MinMax/1
  MinMax/1 -> [Ts]
  Constant9/1 -> MinMax/2
  MinMax1/1 -> [OmegaUp]
  MinMax2/1 -> [OmegaDn]
  [Ts] -> Math Function/1
  Math Function/1 -> Gain/1
  Gain/1 -> MinMax1/2, MinMax2/1
  Constant3/1 -> MinMax1/1
  Constant4/1 -> MinMax2/2
  Product1/1 -> Saturation/1
  Product2/1 -> Saturation1/1

== system My_gfm_battery_sil_12_ConvIGBT_zDomain/My Inverter Controller /My_circuit_controls_A4/virtual damper/Damping HPF ==
  note: Forward integrator
  in : Inport
  Constant2 : Constant  Value=Ts
  Constant3 : Constant  Value=OmegaUp
  Constant4 : Constant  Value=OmegaDn
  Constant9 : Constant  Value=1/20000
  Delay : Delay  DelayLength=1  InitialCondition=0
  Gain : Gain  Gain=1/5
  Math Function : Math  Operator=reciprocal  SignedPower=on
  MinMax : MinMax  Function=max  Inputs=2
  MinMax1 : MinMax  Inputs=2
  MinMax2 : MinMax  Inputs=2
  Product : Product
  Product1 : Product
  Product2 : Product
  Saturation : Saturate  UpperLimit=inf  LowerLimit=0
  Saturation1 : Saturate  UpperLimit=0  LowerLimit=-inf
  Sum : Sum  Inputs=|+-
  Sum1 : Sum  Inputs=|++
  Sum2 : Sum  Inputs=|++
  Sum3 : Sum  Inputs=|+-
  out : Outport  VectorParamsAs1DForOutWhenUnconnected=off
  wires:
  Gain/1 -> MinMax1/2, MinMax2/1
  [Ts] -> Product/1
  [Ts] -> Math Function/1
  Delay/1 -> Sum1/2, Sum/2
  MinMax1/1 -> [OmegaUp]
  Constant9/1 -> MinMax/2
  Sum/1 -> Product2/1, Product1/2
  Math Function/1 -> Gain/1
  Constant4/1 -> MinMax2/2
  Constant2/1 -> MinMax/1
  Saturation/1 -> Sum2/1
  Sum1/1 -> Sum3/2, Delay/1
  Sum2/1 -> Product/2
  MinMax2/1 -> [OmegaDn]
  Product/1 -> Sum1/1
  [OmegaUp] -> Product1/1
  Constant3/1 -> MinMax1/1
  MinMax/1 -> [Ts]
  Product2/1 -> Saturation1/1
  in/1 -> Sum3/1, Sum/1
  Product1/1 -> Saturation/1
  [OmegaDn] -> Product2/2
  Saturation1/1 -> Sum2/2
  Sum3/1 -> out/1

== system My_gfm_battery_sil_12_ConvIGBT_zDomain/My Inverter Controller /My_currentLimiting_B/Current_foldback1/LPF4 ==
  note: Forward integrator
  in : Inport
  Constant : Constant  Value=Ts
  Constant1 : Constant  Value=Ts
  Constant2 : Constant  Value=OmegaUp
  Constant3 : Constant  Value=OmegaUp
  Constant4 : Constant  Value=OmegaDn
  Delay : Delay  DelayLength=1  InitialCondition=0
  Product{,1..4} (5 alike) : Product
  Saturation : Saturate  UpperLimit=inf  LowerLimit=0
  Saturation1 : Saturate  UpperLimit=0  LowerLimit=-inf
  Sum : Sum  Inputs=|++
  Sum1 : Sum  Inputs=|++
  Sum4 : Sum  Inputs=|+-
  out : Outport
  wires:
  Delay/1 -> Sum4/2, Sum/2
  in/1 -> Sum4/1, Product4/2
  Sum4/1 -> Product2/1, Product1/2
  Sum/1 -> out/1, Delay/1
  Saturation/1 -> Sum1/1
  Saturation1/1 -> Sum1/2
  Sum1/1 -> Product/2
  Product/1 -> Sum/1
  Constant/1 -> Product/1
  Constant3/1 -> Product1/1
  Constant4/1 -> Product2/2
  Product1/1 -> Saturation/1
  Product2/1 -> Saturation1/1
  Product4/1 -> Product3/2
  Constant1/1 -> Product3/1
  Constant2/1 -> Product4/1

== system My_gfm_battery_sil_12_ConvIGBT_zDomain/My Inverter Controller /My_currentLimiting_B/RMS_Analyzer/LPF4 ==
  note: Forward integrator
  in : Inport
  Constant : Constant  Value=Ts
  Constant1 : Constant  Value=Ts
  Constant2 : Constant  Value=OmegaUp
  Constant3 : Constant  Value=OmegaUp
  Constant4 : Constant  Value=OmegaDn
  Delay : Delay  DelayLength=1  InitialCondition=0
  Product{,1..4} (5 alike) : Product
  Saturation : Saturate  UpperLimit=inf  LowerLimit=0
  Saturation1 : Saturate  UpperLimit=0  LowerLimit=-inf
  Sum : Sum  Inputs=|++
  Sum1 : Sum  Inputs=|++
  Sum4 : Sum  Inputs=|+-
  out : Outport
  wires:
  Delay/1 -> Sum4/2, Sum/2
  in/1 -> Sum4/1, Product4/2
  Sum4/1 -> Product2/1, Product1/2
  Sum/1 -> out/1, Delay/1
  Saturation/1 -> Sum1/1
  Saturation1/1 -> Sum1/2
  Sum1/1 -> Product/2
  Product/1 -> Sum/1
  Constant/1 -> Product/1
  Constant3/1 -> Product1/1
  Constant4/1 -> Product2/2
  Product1/1 -> Saturation/1
  Product2/1 -> Saturation1/1
  Product4/1 -> Product3/2
  Constant1/1 -> Product3/1
  Constant2/1 -> Product4/1

== system My_gfm_battery_sil_12_ConvIGBT_zDomain/My Inverter Controller /My_currentLimiting_B/RMS_Analyzer1/LPF4 ==
  note: Forward integrator
  in : Inport
  Constant : Constant  Value=Ts
  Constant1 : Constant  Value=Ts
  Constant2 : Constant  Value=OmegaUp
  Constant3 : Constant  Value=OmegaUp
  Constant4 : Constant  Value=OmegaDn
  Delay : Delay  DelayLength=1  InitialCondition=0
  Product{,1..4} (5 alike) : Product
  Saturation : Saturate  UpperLimit=inf  LowerLimit=0
  Saturation1 : Saturate  UpperLimit=0  LowerLimit=-inf
  Sum : Sum  Inputs=|++
  Sum1 : Sum  Inputs=|++
  Sum4 : Sum  Inputs=|+-
  out : Outport
  wires:
  Delay/1 -> Sum4/2, Sum/2
  in/1 -> Sum4/1, Product4/2
  Sum4/1 -> Product2/1, Product1/2
  Sum/1 -> out/1, Delay/1
  Saturation/1 -> Sum1/1
  Saturation1/1 -> Sum1/2
  Sum1/1 -> Product/2
  Product/1 -> Sum/1
  Constant/1 -> Product/1
  Constant3/1 -> Product1/1
  Constant4/1 -> Product2/2
  Product1/1 -> Saturation/1
  Product2/1 -> Saturation1/1
  Product4/1 -> Product3/2
  Constant1/1 -> Product3/1
  Constant2/1 -> Product4/1

== system My_gfm_battery_sil_12_ConvIGBT_zDomain/My Inverter Controller /My_currentLimiting_B/SOGI1/Integrator ==
  in : Inport
  rst : Inport  Port=2
  Constant : Constant  Value=0
  Constant1 : Constant  Value=HiLim
  Constant2 : Constant  Value=LoLim
  Constant3 : Constant  Value=Ts
  Delay : Delay  DelayLength=1  InitialCondition=0
  Logical Operator : Logic  Operator=NOT  AllPortsSameDT=off  OutDataTypeStr=boolean
  Product : Product
  Saturation Dynamic : simulink/Discontinuities/Saturation Dynamic  OutMin=[]  OutMax=[]  OutDataTypeStr=Inherit: Same as second input  OutDataType=fixdt(1, 16)  OutScaling=2^-10  DoSatur=off
  Sum : Sum  Inputs=|++
  Switch : Switch  Criteria=u2 ~= 0  SaturateOnIntegerOverflow=off  InputSameDT=off
  out : Outport
  FB : Outport  Port=2
  wires:
  Delay/1 -> Sum/2, FB/1
  Switch/1 -> Saturation Dynamic/2
  in/1 -> Product/2
  Product/1 -> Sum/1
  Constant3/1 -> Product/1
  Sum/1 -> Switch/1
  Constant/1 -> Switch/3
  rst/1 -> Logical Operator/1
  Logical Operator/1 -> Switch/2
  Saturation Dynamic/1 -> out/1, Delay/1
  Constant1/1 -> Saturation Dynamic/1
  Constant2/1 -> Saturation Dynamic/3

== system My_gfm_battery_sil_12_ConvIGBT_zDomain/My Inverter Controller /My_currentLimiting_B/SOGI1/Integrator1 ==
  in : Inport
  rst : Inport  Port=2
  Constant : Constant  Value=0
  Constant1 : Constant  Value=HiLim
  Constant2 : Constant  Value=LoLim
  Constant3 : Constant  Value=Ts
  Delay : Delay  DelayLength=1  InitialCondition=0
  Logical Operator : Logic  Operator=NOT  AllPortsSameDT=off  OutDataTypeStr=boolean
  Product : Product
  Saturation Dynamic : simulink/Discontinuities/Saturation Dynamic  OutMin=[]  OutMax=[]  OutDataTypeStr=Inherit: Same as second input  OutDataType=fixdt(1, 16)  OutScaling=2^-10  DoSatur=off
  Sum : Sum  Inputs=|++
  Switch : Switch  Criteria=u2 ~= 0  SaturateOnIntegerOverflow=off  InputSameDT=off
  out : Outport
  FB : Outport  Port=2
  wires:
  Delay/1 -> Sum/2, FB/1
  Switch/1 -> Saturation Dynamic/2
  in/1 -> Product/2
  Product/1 -> Sum/1
  Constant3/1 -> Product/1
  Sum/1 -> Switch/1
  Constant/1 -> Switch/3
  rst/1 -> Logical Operator/1
  Logical Operator/1 -> Switch/2
  Saturation Dynamic/1 -> out/1, Delay/1
  Constant1/1 -> Saturation Dynamic/1
  Constant2/1 -> Saturation Dynamic/3

== system My_gfm_battery_sil_12_ConvIGBT_zDomain/My Inverter Controller /My_machineModel_A1/excitation/LPF ==
  In : Inport
  Integrator : Integrator
  Sum3 : Sum  Inputs=|+-
  wExciter : Gain  Gain=wExciter
  Out : Outport
  wires:
  Integrator/1 -> Out/1, Sum3/2
  Sum3/1 -> wExciter/1
  In/1 -> Sum3/1
  wExciter/1 -> Integrator/1

== system My_gfm_battery_sil_12_ConvIGBT_zDomain/My Inverter Controller /My_machineModel_A1/excitation/assymmetric filter1 ==
  note: The saturation block is configured to cause a rapid rise, but much slow drop in output.
  in : Inport
  Gain1 : Gain  Gain=2
  Integrator : Integrator
  Saturation1 : Saturate  UpperLimit=VllRated  LowerLimit=-0.02 * VllRated
  Sum3 : Sum  Inputs=|+-
  out : Outport
  wires:
  Saturation1/1 -> Integrator/1
  Gain1/1 -> Saturation1/1
  in/1 -> Sum3/1
  Sum3/1 -> Gain1/1
  Integrator/1 -> Sum3/2, out/1

== system My_gfm_battery_sil_12_ConvIGBT_zDomain/My Inverter Controller /My_machineModel_A1/excitation/modulator ==
  cmd : Inport
  osc : Inport  Port=2
  Complex to Real-Imag : ComplexToRealImag
  Complex to Real-Imag1 : ComplexToRealImag
  Gain : Gain  Gain=sqrt(2)
  Product1 : Product
  Product2 : Product
  Sum1 : Sum  Inputs=|+-
  ref : Outport
  wires:
  osc/1 -> Gain/1
  Complex to Real-Imag/1 -> Product2/2
  Product2/1 -> Sum1/1
  Sum1/1 -> ref/1  "i"
  Gain/1 -> Complex to Real-Imag/1
  Complex to Real-Imag/2 -> Product1/2
  Product1/1 -> Sum1/2
  cmd/1 -> Complex to Real-Imag1/1
  Complex to Real-Imag1/1 -> Product2/1
  Complex to Real-Imag1/2 -> Product1/1

== system My_gfm_battery_sil_12_ConvIGBT_zDomain/My Inverter Controller /My_machineModel_A1/governer/LPF(DamperDecoupler) limited  ==
  In : Inport
  1/tau_damp : Gain  Gain=1/0.3
  Integrator : Integrator  LimitOutput=on  UpperSaturationLimit=1.2*SRated  LowerSaturationLimit=-1.2*SRated
  Sum3 : Sum  Inputs=|+-
  Out : Outport
  wires:
  Integrator/1 -> Out/1, Sum3/2
  Sum3/1 -> 1/tau_damp/1
  In/1 -> Sum3/1
  1/tau_damp/1 -> Integrator/1

== system My_gfm_battery_sil_12_ConvIGBT_zDomain/My Inverter Controller /My_machineModel_A1/governer/synchronizer ==
  note: Why?
  note: Big Range?
  note: prevent it from acting during typical faults
  note: Prevent loss of sync at low voltage events, using asym filter to traget long extended low voltage events
  note: Keeps the machine spining in synchronize while machine is disabled, disabling the machine means
  note: Why?
  Vq : Inport
  Vt : Inport  Port=2
  machine_enabled : Inport  Port=3
  Constant : Constant
  Gain : Gain  Gain=SRated
  Gain2 : Gain  Gain=1/VllRated
  HPF : Subsystem
  Product1 : Product
  Saturation : Saturate  UpperLimit=1  LowerLimit=0
  Sum : Sum  Inputs=|++
  Sum2 : Sum  Inputs=|+-
  Switch : Switch  Criteria=u2 > Threshold  SaturateOnIntegerOverflow=off  InputSameDT=off
  Transfer Fcn : TransferFcn  Commented=on  Numerator=[(2 * pi * 50) 0]  Denominator=[1, (2*pi*50)]
  assymmetric filter1 : Subsystem
  gain : Gain  Gain=2*pi*50
  kFastSync : Gain
  kSync : Gain  Gain=20
  pSyncLimit : Saturate  UpperLimit=3  LowerLimit=-3
  syncFadeGain : Gain  Gain=4
  syncFadeThreshold : Constant  Value=0.2
  to_pu : Gain  Gain=1 / VllRated
  p_sync_pu : Outport
  wires:
  to_pu/1 -> Sum2/2
  Vt/1 -> assymmetric filter1/1(in)
  assymmetric filter1/1(out) -> to_pu/1
  pSyncLimit/1 -> Gain/1
  kSync/1 -> Sum/1
  Sum/1 -> pSyncLimit/1
  Product1/1 -> p_sync_pu/1
  Constant/1 -> Switch/3
  Sum2/1 -> syncFadeGain/1
  machine_enabled/1 -> Switch/2
  syncFadeGain/1 -> Saturation/1
  Saturation/1 -> Switch/1
  syncFadeThreshold/1 -> Sum2/1
  Switch/1 -> Product1/2
  Gain2/1 -> kFastSync/1, kSync/1
  Vq/1 -> Gain2/1
  Gain/1 -> Product1/1  "p_sync"
  kFastSync/1 -> HPF/1(in)
  HPF/1(out) -> gain/1
  gain/1 -> Sum/2

== system My_gfm_battery_sil_12_ConvIGBT_zDomain/My Inverter Controller /My_machineModel_A1/governer1/LPF(DamperDecoupler) - limited ==
  In1 : Inport
  Integrator : Integrator  LimitOutput=on  UpperSaturationLimit=1.2*SRated  LowerSaturationLimit=-1.2*SRated
  Sum3 : Sum  Inputs=|+-
  wDamperDecoupler : Gain  Gain=1/0.3
  Out1 : Outport
  wires:
  Integrator/1 -> Out1/1, Sum3/2
  Sum3/1 -> wDamperDecoupler/1
  wDamperDecoupler/1 -> Integrator/1
  In1/1 -> Sum3/1
